simulink model "WBR_control"  (R2021b)
settings: Solver=ode4  StartTime=0.0  StopTime=12  FixedStep=1e-4  RelTol=1e-3
undefined symbols (not defined in the file): leg_controller, leg_l1, leg_l2, leg_model, leg_r1, leg_r2, locomotion_controller, param, sigbuilder_block, wheel_l, wheel_r, X, Y, Z
libraries: sm_lib x110, nesl_utility x29, slpidlib x2
(part 1 of 4)
settings Model: SimulationMode=accelerator  Creator=thinkpad  LastModifiedBy=thinkpad
settings OptimizationCC: DefaultUnderspecifiedDataType=single

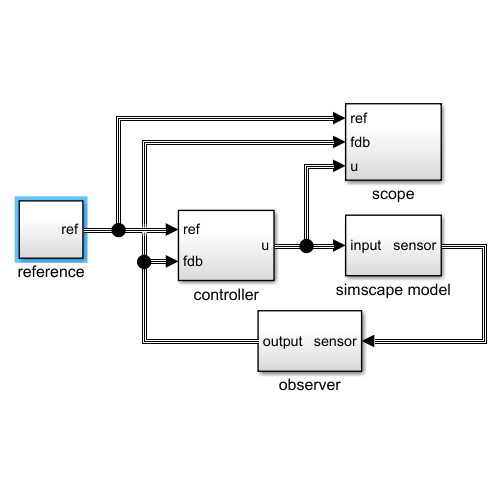
[thumbnail: Simulink's stored preview of the top-level diagram]
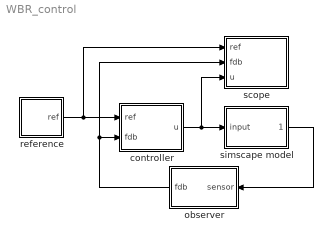
== system WBR_control ==
  controller : Subsystem
  observer : Subsystem
  reference : Subsystem
  scope : Subsystem
  simscape model : Subsystem
  wires:
  reference/1(ref) -> scope/1(ref), controller/1(ref)
  controller/1(u) -> simscape model/1(input), scope/3(u)
  simscape model/1(sensor) -> observer/1(sensor)
  observer/1(fdb) -> controller/2(fdb), scope/2(fdb)

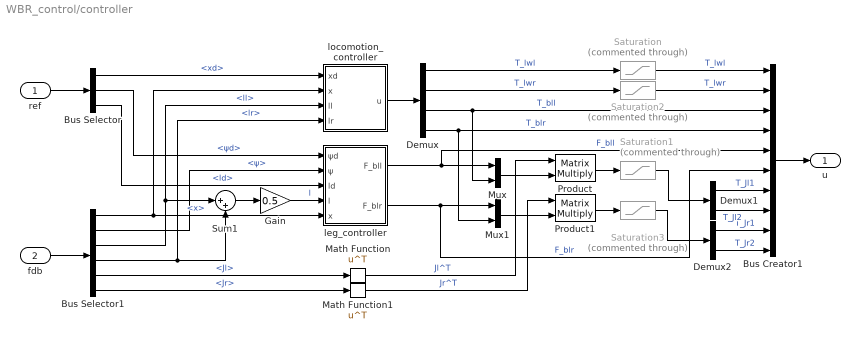
== system WBR_control/controller ==
  ref : Inport
  fdb : Inport  Port=2
  Bus Creator1 : BusCreator  Inputs=10
  Bus Selector : BusSelector  OutputSignals=xd,ψd,ld
  Bus Selector1 : BusSelector  OutputSignals=x,ψ,ll,lr,Jl,Jr
  Demux : Demux
  Demux1 : Demux  Outputs=2
  Demux2 : Demux  Outputs=2
  Gain : Gain  Gain=0.5
  Math Function : Math  Operator=transpose  SaturateOnIntegerOverflow=on
  Math Function1 : Math  Operator=transpose  SaturateOnIntegerOverflow=on
  Mux : Mux  Inputs=2
  Mux1 : Mux  Inputs=2
  Product : Product  Multiplication=Matrix(*)
  Product1 : Product  Multiplication=Matrix(*)
  Saturation : Saturate  Commented=through  UpperLimit=4  LowerLimit=-4
  Saturation1 : Saturate  Commented=through  UpperLimit=[35,35]  LowerLimit=-[35,35]
  Saturation2 : Saturate  Commented=through  UpperLimit=4  LowerLimit=-4
  Saturation3 : Saturate  Commented=through  UpperLimit=[35,35]  LowerLimit=-[35,35]
  Sum1 : Sum  Inputs=|++
  leg_controller : Subsystem
  locomotion_controller : Subsystem
  u : Outport
  wires:
  Bus Selector/1 -> locomotion_controller/1(xd)  "<xd>"
  locomotion_controller/1(u) -> Demux/1
  Demux/1 -> Saturation/1  "T_lwl"
  leg_controller/1(F_bll) -> Bus Creator1/5, Mux/1  "F_bll"
  Bus Selector/2 -> leg_controller/1(ψd)  "<ψd>"
  Bus Selector/3 -> leg_controller/3(ld)  "<ld>"
  Mux/1 -> Product/2
  Product/1 -> Saturation1/1
  ref/1 -> Bus Selector/1
  fdb/1 -> Bus Selector1/1
  Bus Selector1/1 -> locomotion_controller/2(x), leg_controller/5(x)  "<x>"
  Bus Selector1/3 -> locomotion_controller/3(ll), Sum1/1  "<ll>"
  Bus Selector1/4 -> locomotion_controller/4(lr), Sum1/2  "<lr>"
  Bus Selector1/5 -> Math Function/1  "<Jl>"
  Math Function/1 -> Product/1  "Jl^T"
  Demux/2 -> Saturation2/1  "T_lwr"
  Sum1/1 -> Gain/1
  Gain/1 -> leg_controller/4(l)  "l"
  Bus Selector1/6 -> Math Function1/1  "<Jr>"
  Demux/3 -> Mux/2, Bus Creator1/3  "T_bll"
  Demux/4 -> Mux1/2, Bus Creator1/4  "T_blr"
  leg_controller/2(F_blr) -> Bus Creator1/6, Mux1/1  "F_blr"
  Math Function1/1 -> Product1/1  "Jr^T"
  Mux1/1 -> Product1/2
  Product1/1 -> Saturation3/1
  Saturation1/1 -> Demux1/1
  Saturation3/1 -> Demux2/1
  Saturation2/1 -> Bus Creator1/2  "T_lwr"
  Saturation/1 -> Bus Creator1/1  "T_lwl"
  Demux2/1 -> Bus Creator1/9  "T_Jr1"
  Demux2/2 -> Bus Creator1/10  "T_Jr2"
  Demux1/1 -> Bus Creator1/7  "T_Jl1"
  Demux1/2 -> Bus Creator1/8  "T_Jl2"
  Bus Creator1/1 -> u/1
  Bus Selector1/2 -> leg_controller/2(ψ)  "<ψ>"

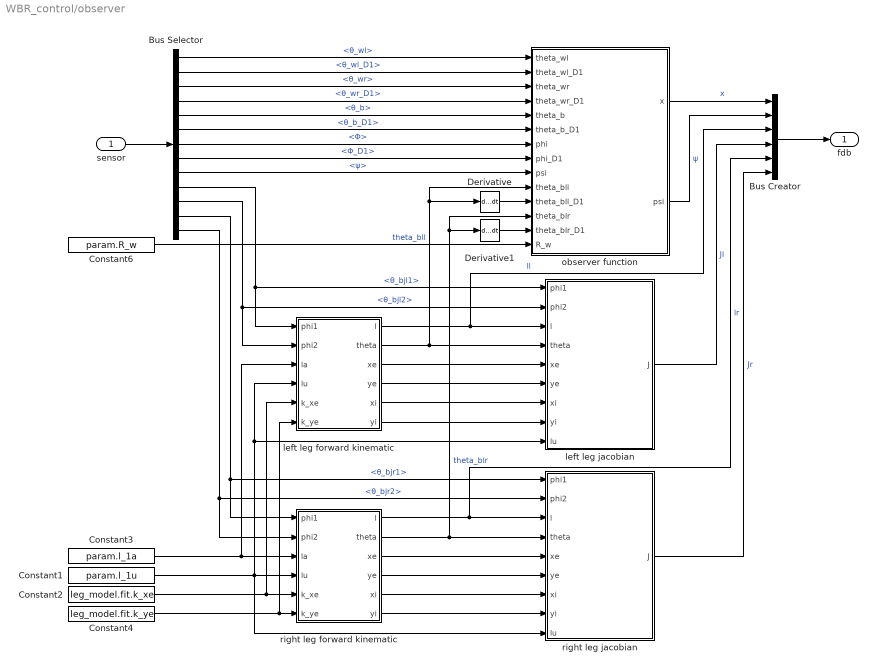
== system WBR_control/observer ==
  sensor : Inport
  Bus Creator : BusCreator  Inputs=6
  Bus Selector : BusSelector  OutputSignals=θ_wl,θ_wl_D1,θ_wr,θ_wr_D1,θ_b,θ_b_D1,Φ,Φ_D1,ψ,θ_bjl1,θ_bjl2,θ_bjr1,θ_bjr2
  Constant1 : Constant  Value=param.l_1u
  Constant2 : Constant  Value=leg_model.fit.k_xe
  Constant3 : Constant  Value=param.l_1a
  Constant4 : Constant  Value=leg_model.fit.k_ye
  Constant6 : Constant  Value=param.R_w
  Derivative : Derivative
  Derivative1 : Derivative
  left leg forward kinematic : MATLAB Function  TreatAsAtomicUnit=on
  left leg jacobian : MATLAB Function  TreatAsAtomicUnit=on
  observer function : MATLAB Function  TreatAsAtomicUnit=on
  right leg forward kinematic : MATLAB Function  TreatAsAtomicUnit=on
  right leg jacobian : MATLAB Function  TreatAsAtomicUnit=on
  fdb : Outport
  wires:
  sensor/1 -> Bus Selector/1
  right leg forward kinematic/3(xe) -> right leg jacobian/5(xe)
  right leg forward kinematic/4(ye) -> right leg jacobian/6(ye)
  right leg forward kinematic/5(xi) -> right leg jacobian/7(xi)
  right leg forward kinematic/6(yi) -> right leg jacobian/8(yi)
  right leg forward kinematic/1(l) -> right leg jacobian/3(l), Bus Creator/5  "lr"
  left leg forward kinematic/1(l) -> Bus Creator/3, left leg jacobian/3(l)  "ll"
  Bus Creator/1 -> fdb/1
  right leg jacobian/1(J) -> Bus Creator/6  "Jr"
  Bus Selector/1 -> observer function/1(theta_wl)  "<θ_wl>"
  Bus Selector/2 -> observer function/2(theta_wl_D1)  "<θ_wl_D1>"
  Bus Selector/3 -> observer function/3(theta_wr)  "<θ_wr>"
  Bus Selector/4 -> observer function/4(theta_wr_D1)  "<θ_wr_D1>"
  Bus Selector/5 -> observer function/5(theta_b)  "<θ_b>"
  Bus Selector/6 -> observer function/6(theta_b_D1)  "<θ_b_D1>"
  Bus Selector/7 -> observer function/7(phi)  "<Φ>"
  Bus Selector/8 -> observer function/8(phi_D1)  "<Φ_D1>"
  left leg jacobian/1(J) -> Bus Creator/4  "Jl"
  observer function/1(x) -> Bus Creator/1  "x"
  observer function/2(psi) -> Bus Creator/2  "ψ"
  Bus Selector/9 -> observer function/9("psi ")  "<ψ>"
  Bus Selector/10 -> left leg forward kinematic/1(phi1), left leg jacobian/1(phi1)  "<θ_bjl1>"
  Bus Selector/11 -> left leg forward kinematic/2(phi2), left leg jacobian/2(phi2)  "<θ_bjl2>"
  left leg forward kinematic/2(theta) -> observer function/10(theta_bll), Derivative/1, left leg jacobian/4(theta)  "theta_bll"
  Derivative/1 -> observer function/11(theta_bll_D1)
  Bus Selector/12 -> right leg jacobian/1(phi1), right leg forward kinematic/1(phi1)  "<θ_bjr1>"
  Bus Selector/13 -> right leg jacobian/2(phi2), right leg forward kinematic/2(phi2)  "<θ_bjr2>"
  right leg forward kinematic/2(theta) -> right leg jacobian/4(theta), observer function/12(theta_blr), Derivative1/1  "theta_blr"
  Derivative1/1 -> observer function/13(theta_blr_D1)
  left leg forward kinematic/4(ye) -> left leg jacobian/6(ye)
  left leg forward kinematic/5(xi) -> left leg jacobian/7(xi)
  left leg forward kinematic/6(yi) -> left leg jacobian/8(yi)
  left leg forward kinematic/3(xe) -> left leg jacobian/5(xe)
  Constant3/1 -> left leg forward kinematic/3(la), right leg forward kinematic/3(la)
  Constant1/1 -> right leg forward kinematic/4(lu), right leg jacobian/9(lu), left leg forward kinematic/4(lu), left leg jacobian/9(lu)
  Constant2/1 -> left leg forward kinematic/5(k_xe), right leg forward kinematic/5(k_xe)
  Constant4/1 -> left leg forward kinematic/6(k_ye), right leg forward kinematic/6(k_ye)
  Constant6/1 -> observer function/14(R_w)

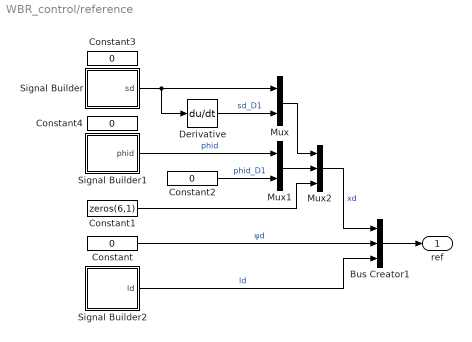
== system WBR_control/reference ==
  Bus Creator1 : BusCreator  Inputs=3
  Constant{,2..4} (4 alike) : Constant  Value=0
  Constant1 : Constant  Value=zeros(6,1)
  Derivative : Derivative
  Mux : Mux  Inputs=2
  Mux1 : Mux  Inputs=2
  Mux2 : Mux  Inputs=3
  Signal Builder : Subsystem  Tag=STV Subsys  LoadFcn=sigbuilder_block('load');  StartFcn=sigbuilder_block('start');  StopFcn=sigbuilder_block('stop');  ClipboardFcn=sigbuilder_block('clipboard');  mask(Sigbuilder block){tuvar=[0:10]}
      mask help: Simulink:masks:SigbuilderBlock_MD
      mask init:
      | if ~strcmp(get_param(bdroot(gcbh),'SimulationStatus'),'stopped') tuvar = sigbuilder_block('maskInit'); end
      settings: CopyFcn=sigbuilder_block('copy');  DeleteFcn=sigbuilder_block('delete');  ModelCloseFcn=sigbuilder_block('modelClose');  PreSaveFcn=sigbuilder_block('preSave');  PauseFcn=sigbuilder_block('pause');  ContinueFcn=sigbuilder_block('continue');  NameChangeFcn=sigbuilder_block('namechange');  OpenFcn=sigbuilder_block('open',[427.2 154.8 550.8 400.2 ]);  CloseFcn=sigbuilder_block('close');
      mask Display: plot(0, 0, 100, 100,[2, 2, 32, 32, 2], [68, 8, 8, 68, 68],[32, 2], [38, 38], [32, 19, 2],[53, 60, 44], [32, 17, 17, 2],[16, 16, 31, 31]);txt = getActiveGroup(gcbh);text(2, 100, txt,'verticalAlignment', 'top');
  Signal Builder1 : Subsystem  Tag=STV Subsys  LoadFcn=sigbuilder_block('load');  StartFcn=sigbuilder_block('start');  StopFcn=sigbuilder_block('stop');  ClipboardFcn=sigbuilder_block('clipboard');  mask(Sigbuilder block){tuvar=[0:10]}
      mask help: Simulink:masks:SigbuilderBlock_MD
      mask init:
      | if ~strcmp(get_param(bdroot(gcbh),'SimulationStatus'),'stopped') tuvar = sigbuilder_block('maskInit'); end
      settings: CopyFcn=sigbuilder_block('copy');  DeleteFcn=sigbuilder_block('delete');  ModelCloseFcn=sigbuilder_block('modelClose');  PreSaveFcn=sigbuilder_block('preSave');  PauseFcn=sigbuilder_block('pause');  ContinueFcn=sigbuilder_block('continue');  NameChangeFcn=sigbuilder_block('namechange');  OpenFcn=sigbuilder_block('open',[427.2 154.8 550.8 400.2 ]);  CloseFcn=sigbuilder_block('close');
      mask Display: plot(0, 0, 100, 100,[2, 2, 32, 32, 2], [68, 8, 8, 68, 68],[32, 2], [38, 38], [32, 19, 2],[53, 60, 44], [32, 17, 17, 2],[16, 16, 31, 31]);txt = getActiveGroup(gcbh);text(2, 100, txt,'verticalAlignment', 'top');
  Signal Builder2 : Subsystem  Tag=STV Subsys  LoadFcn=sigbuilder_block('load');  StartFcn=sigbuilder_block('start');  StopFcn=sigbuilder_block('stop');  ClipboardFcn=sigbuilder_block('clipboard');  mask(Sigbuilder block){tuvar=[0:10]}
      mask help: Simulink:masks:SigbuilderBlock_MD
      mask init:
      | if ~strcmp(get_param(bdroot(gcbh),'SimulationStatus'),'stopped') tuvar = sigbuilder_block('maskInit'); end
      settings: CopyFcn=sigbuilder_block('copy');  DeleteFcn=sigbuilder_block('delete');  ModelCloseFcn=sigbuilder_block('modelClose');  PreSaveFcn=sigbuilder_block('preSave');  PauseFcn=sigbuilder_block('pause');  ContinueFcn=sigbuilder_block('continue');  NameChangeFcn=sigbuilder_block('namechange');  OpenFcn=sigbuilder_block('open',[427.2 154.8 550.8 400.2 ]);  CloseFcn=sigbuilder_block('close');
      mask Display: plot(0, 0, 100, 100,[2, 2, 32, 32, 2], [68, 8, 8, 68, 68],[32, 2], [38, 38], [32, 19, 2],[53, 60, 44], [32, 17, 17, 2],[16, 16, 31, 31]);txt = getActiveGroup(gcbh);text(2, 100, txt,'verticalAlignment', 'top');
  ref : Outport
  wires:
  Mux2/1 -> Bus Creator1/1  "xd"
  Constant1/1 -> Mux2/3
  Signal Builder/1(sd) -> Derivative/1, Mux/1
  Bus Creator1/1 -> ref/1
  Constant2/1 -> Mux1/2  "phid_D1"
  Constant/1 -> Bus Creator1/2  "ψd"
  Mux/1 -> Mux2/1
  Mux1/1 -> Mux2/2
  Signal Builder2/1(ld) -> Bus Creator1/3  "ld"
  Derivative/1 -> Mux/2  "sd_D1"
  Signal Builder1/1(phid) -> Mux1/1  "phid"

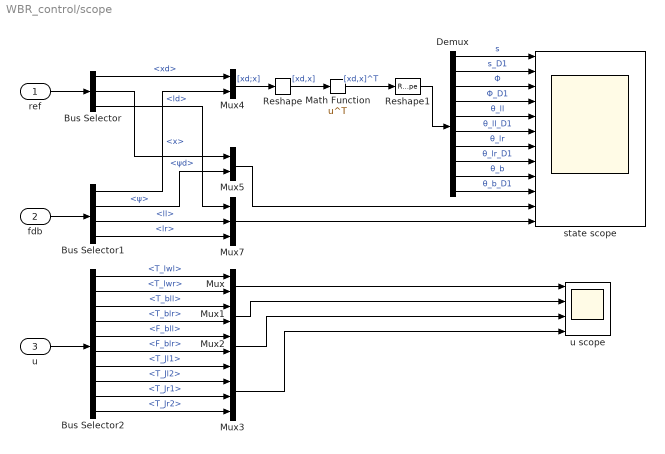
== system WBR_control/scope ==
  ref : Inport
  fdb : Inport  Port=2
  u : Inport  Port=3
  Bus Selector : BusSelector  OutputSignals=xd,ψd,ld
  Bus Selector1 : BusSelector  OutputSignals=x,ψ,ll,lr
  Bus Selector2 : BusSelector  OutputSignals=T_lwl,T_lwr,T_bll,T_blr,F_bll,F_blr,T_Jl1,T_Jl2,T_Jr1,T_Jr2
  Demux : Demux  Outputs=10
  Math Function : Math  Operator=transpose  SaturateOnIntegerOverflow=on
  Mux{,1..2,4..5} (5 alike) : Mux  Inputs=2
  Mux3 : Mux
  Mux7 : Mux  Inputs=3
  Reshape : Reshape  OutputDimensionality=Customize  OutputDimensions=[10,2]
  Reshape1 : Reshape
  state scope : Scope  NumInputPorts=12
  u scope : Scope  NumInputPorts=4
  wires:
  ref/1 -> Bus Selector/1
  fdb/1 -> Bus Selector1/1
  u/1 -> Bus Selector2/1
  Bus Selector2/1 -> Mux/1  "<T_lwl>"
  Bus Selector2/2 -> Mux/2  "<T_lwr>"
  Bus Selector2/3 -> Mux1/1  "<T_bll>"
  Bus Selector2/4 -> Mux1/2  "<T_blr>"
  Bus Selector2/5 -> Mux2/1  "<F_bll>"
  Bus Selector2/6 -> Mux2/2  "<F_blr>"
  Bus Selector2/7 -> Mux3/1  "<T_Jl1>"
  Bus Selector2/8 -> Mux3/2  "<T_Jl2>"
  Bus Selector2/9 -> Mux3/3  "<T_Jr1>"
  Bus Selector2/10 -> Mux3/4  "<T_Jr2>"
  Mux3/1 -> u scope/4
  Mux2/1 -> u scope/3
  Mux1/1 -> u scope/2
  Mux/1 -> u scope/1
  Bus Selector1/1 -> Mux4/2  "<x>"
  Bus Selector/1 -> Mux4/1  "<xd>"
  Bus Selector/2 -> Mux5/1  "<ψd>"
  Bus Selector/3 -> Mux7/1  "<ld>"
  Bus Selector1/2 -> Mux5/2  "<ψ>"
  Bus Selector1/3 -> Mux7/2  "<ll>"
  Bus Selector1/4 -> Mux7/3  "<lr>"
  Mux4/1 -> Reshape/1  "[xd;x]"
  Mux5/1 -> state scope/11
  Mux7/1 -> state scope/12
  Reshape/1 -> Math Function/1  "[xd,x]"
  Math Function/1 -> Reshape1/1  "[xd,x]^T"
  Reshape1/1 -> Demux/1
  Demux/1 -> state scope/1  "s"
  Demux/2 -> state scope/2  "s_D1"
  Demux/3 -> state scope/3  "Φ"
  Demux/4 -> state scope/4  "Φ_D1"
  Demux/6 -> state scope/6  "θ_ll_D1"
  Demux/5 -> state scope/5  "θ_ll"
  Demux/7 -> state scope/7  "θ_lr"
  Demux/8 -> state scope/8  "θ_lr_D1"
  Demux/10 -> state scope/10  "θ_b_D1"
  Demux/9 -> state scope/9  "θ_b"

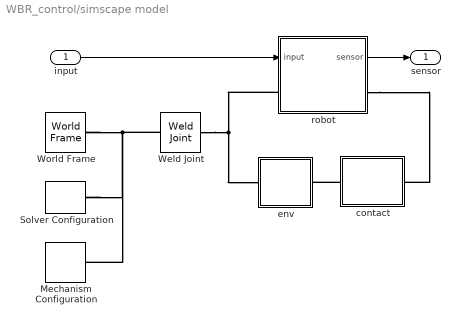
== system WBR_control/simscape model ==
  input : Inport
  Mechanism Configuration : sm_lib/Utilities/Mechanism Configuration  UniformGravity=Constant  GravityVector=[0 0 -9.81]  GravityUnits=m/s^2  LinearizationDelta=0.001  JointModeTransitionNonlinearIterations=2
  Solver Configuration : nesl_utility/Solver Configuration  PhysicalDomain=network_engine_domain  SubClassName=solver  LeftPortType=input  RightPortType=generic  Tones=[]  Harmonics=[]  SimulateNoise=off  Profile=off  UseLocalSampling=off  EnableSwitchedLinearOptims=on  FrequencyDomain=off  UseCCode=off  RelTol=0.001  AbsTol=1e-06  MinStep=1e-09  ToWorkspace=off  RevertToSquareIcSolve=off  NumHomotopyIterations=100  PhasorMode=off  PhasorModeNumHarmonics=1  DoDC=off  ResidualTolerance=1e-09  UseLocalSolver=off  LocalSolverChoice=NE_BACKWARD_EULER_ADVANCER  LocalSolverSampleTime=0.001  DoFixedCost=off  MaxNonlinIter=3  MaxModeIter=2  ComputeImpulses=off  ImpulseIterations=2  LinearAlgebra=Sparse  EquationFormulation=NE_TIME_EF  DelaysMemoryBudget=1024  AutomaticFiltering=on  FilteringTimeConstant=0.001  PartitionStorageMethod=AS_NEEDED  PartitionMemoryBudget=1024  PartitionMethod=FAST
      settings: SourceProductBaseCode=PW,SS
  Weld Joint : sm_lib/Joints/Weld Joint  JointMode=Normal  SenseConstraintForce=off  SenseConstraintForceX=off  SenseConstraintForceY=off  SenseConstraintForceZ=off  SenseConstraintTorque=off  SenseConstraintTorqueX=off  SenseConstraintTorqueY=off  SenseConstraintTorqueZ=off  SenseTotalForce=off  SenseTotalForceX=off  SenseTotalForceY=off  SenseTotalForceZ=off  SenseTotalTorque=off  SenseTotalTorqueX=off  SenseTotalTorqueY=off  SenseTotalTorqueZ=off  CompositeWrenchDir=FollowerOnBase  CompositeWrenchFrame=BaseFrame
  World Frame : sm_lib/Frames and Transforms/World Frame
  contact : Subsystem
      settings: PortSchema="{\"entries\":[{\"content\":{\"sides\":[{\"content\":{\"connectorIds\":[]},\"type\":\"ConnectorPlacement.EquallySpacedRectSide\",\"uuid\":\"948d884d-a2bb-4982-bec2-8891ab05edb1\"},{\"content\":{\"connectorIds\":[],\"side\":\"RIGHT\"},\"type\":\"ConnectorPlacement.EquallySpacedRectSide\",\"uuid\":\"1ab48329-b8c1-41fb-bc52-c8a32a07fc10\"},{\"content\":{\"connectorIds\":[\"LConn1\"],\"side\":\"TOP\"},\"type\":\"ConnectorPlacement.EquallySpacedRectSide\",\"uuid\":\"2430d379-17bc-45a7-9277-8300fd306697\"},{\"content\":{\"connectorIds\":[\"RConn1\"],\"side\":\"BOTTOM\"},\"type\":\"ConnectorPlacement.EquallySpacedRectSide\",\"uuid\":\"c2c22df6-47ef-4364-9ed6-2fe5d2ebd561\"}]},\"type\":\"ConnectorPlacement.EquallySpacedConnector\",\"uuid\":\"bd96c317-3050-474a-affa-ffce42783eb1\"}],\"packageUris\":[\"http://schema.mathworks.com/mf0/Connector/R2020b\"],\"version\":\"1.0\"}"
  env : Subsystem
  robot : Subsystem
  sensor : Outport
  wires:
  input/1 -> robot/1(input)
  robot/1(sensor) -> sensor/1
  connections:
  World Frame/RConn1 -- Solver Configuration/RConn1 -- Mechanism Configuration/RConn1 -- Weld Joint/LConn1
  contact/RConn1 -- env/RConn1
  Weld Joint/RConn1 -- env/LConn1 -- robot/LConn1
  robot/RConn1 -- contact/LConn1

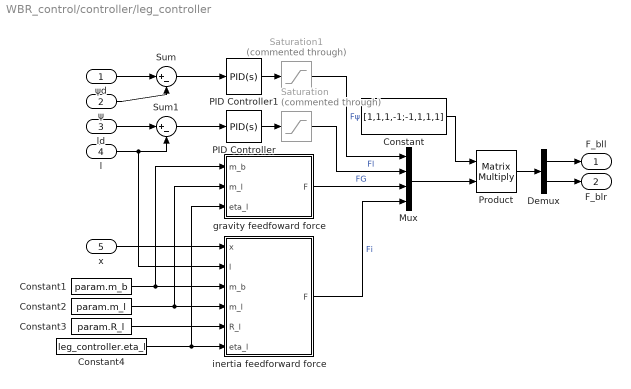
== system WBR_control/controller/leg_controller ==
  ψd : Inport
  ψ : Inport  Port=2
  ld : Inport  Port=3
  l : Inport  Port=4
  x : Inport  Port=5
  Constant : Constant  Value=[1,1,1,-1;-1,1,1,1]
  Constant1 : Constant  Value=param.m_b
  Constant2 : Constant  Value=param.m_l
  Constant3 : Constant  Value=param.R_l
  Constant4 : Constant  Value=leg_controller.eta_l
  Demux : Demux  Outputs=2
  Mux : Mux
  PID Controller : slpidlib/PID Controller  Controller=PID  Form=Parallel  TimeDomain=Continuous-time  UseExternalTs=off  SampleTime=-1  IntegratorMethod=Forward Euler  FilterMethod=Forward Euler  ControllerParametersSource=internal  P=leg_controller.l.kp  I=leg_controller.l.ki  D=leg_controller.l.kd  UseFilter=on  N=100  TunerSelectOption=Transfer Function Based (PID Tuner App)  InitialConditionSource=internal  InitialConditionForIntegrator=0  InitialConditionForFilter=0  DifferentiatorICPrevScaledInput=0  ExternalReset=none  TrackingMode=off  Kt=1  LimitOutput=off  SatLimitsSource=internal  UpperSaturationLimit=inf  LowerSaturationLimit=-inf  LinearizeAsGain=on  AntiWindupMode=none  Kb=1  POutMin=[]  POutMax=[]  IOutMin=[]  IOutMax=[]  DOutMin=[]  DOutMax=[]  NOutMin=[]  NOutMax=[]  SumOutMin=[]  SumOutMax=[]  SaturationOutMin=[]  SaturationOutMax=[]  PParamMin=[]  PParamMax=[]  IParamMin=[]  IParamMax=[]  DParamMin=[]  DParamMax=[]  NParamMin=[]  NParamMax=[]  KbParamMin=[]  KbParamMax=[]  KtParamMin=[]  KtParamMax=[]  KbOutMin=[]  KbOutMax=[]  KtOutMin=[]  KtOutMax=[]  IntegratorOutMin=[]  IntegratorOutMax=[]  FilterOutMin=[]  FilterOutMax=[]  SumI1OutMin=[]  SumI1OutMax=[]  SumI2OutMin=[]  SumI2OutMax=[]  SumI3OutMin=[]  SumI3OutMax=[]  SumI4OutMin=[]  SumI4OutMax=[]  SumDOutMin=[]  SumDOutMax=[]  DifferentiatorOutMin=[]  DifferentiatorOutMax=[]  FilterDiffOutCoefMin=[]  FilterDiffOutCoefMax=[]  ReciprocalOutMin=[]  ReciprocalOutMax=[]  SumDenOutMin=[]  SumDenOutMax=[]  SumNumOutMin=[]  SumNumOutMax=[]  DivideOutMin=[]  DivideOutMax=[]  UdiffTsProdOutMin=[]  UdiffTsProdOutMax=[]  NTsProdOutMin=[]  NTsProdOutMax=[]  UintegralTsProdOutMin=[]  UintegralTsProdOutMax=[]  UngainTsProdOutMin=[]  UngainTsProdOutMax=[]  IntegratorContinuousStateAttributes=''  IntegratorStateMustResolveToSignalObject=off  IntegratorRTWStateStorageClass=Auto  FilterContinuousStateAttributes=''  FilterStateMustResolveToSignalObject=off  FilterRTWStateStorageClass=Auto  ParallelPVariant=InternalParameters  IdealPVariant=Disabled  IVariant=InternalParameters  DVariant=InternalParameters  IntegratorVariant=Continuous  SatVariant=Disabled  AWVariant=Passthrough  PCopyVariant=Disabled  TRVariant=Disabled  FdbkBlocksVariant=Forward  IdealPFdbkVariant=Disabled  SatFdbkVariant=Disabled  DerivativeFilterVariant=ContFilter  NVariant=InternalParameters  NCopyVariant=Disabled  FilterICVariant=InternalICsFilter  IntegratorICVariant=InternalICs  ExternalResetVariant=Disabled  TRSumVariant=Passthrough  SumFdbkVariant=Disabled  SumVariant=Sum_PID  TsampFilterVariant=InternalTs  TsampNgainVariant=Passthrough  TsampIntegralVariant=Passthrough  ExternalSaturationOutDataTypeStr=Inherit: Same as second input
  PID Controller1 : slpidlib/PID Controller  Controller=PID  Form=Parallel  TimeDomain=Continuous-time  UseExternalTs=off  SampleTime=-1  IntegratorMethod=Forward Euler  FilterMethod=Forward Euler  ControllerParametersSource=internal  P=leg_controller.psi.kp  I=leg_controller.psi.ki  D=leg_controller.psi.kd  UseFilter=on  N=100  TunerSelectOption=Transfer Function Based (PID Tuner App)  InitialConditionSource=internal  InitialConditionForIntegrator=0  InitialConditionForFilter=0  DifferentiatorICPrevScaledInput=0  ExternalReset=none  TrackingMode=off  Kt=1  LimitOutput=off  SatLimitsSource=internal  UpperSaturationLimit=inf  LowerSaturationLimit=-inf  LinearizeAsGain=on  AntiWindupMode=none  Kb=1  POutMin=[]  POutMax=[]  IOutMin=[]  IOutMax=[]  DOutMin=[]  DOutMax=[]  NOutMin=[]  NOutMax=[]  SumOutMin=[]  SumOutMax=[]  SaturationOutMin=[]  SaturationOutMax=[]  PParamMin=[]  PParamMax=[]  IParamMin=[]  IParamMax=[]  DParamMin=[]  DParamMax=[]  NParamMin=[]  NParamMax=[]  KbParamMin=[]  KbParamMax=[]  KtParamMin=[]  KtParamMax=[]  KbOutMin=[]  KbOutMax=[]  KtOutMin=[]  KtOutMax=[]  IntegratorOutMin=[]  IntegratorOutMax=[]  FilterOutMin=[]  FilterOutMax=[]  SumI1OutMin=[]  SumI1OutMax=[]  SumI2OutMin=[]  SumI2OutMax=[]  SumI3OutMin=[]  SumI3OutMax=[]  SumI4OutMin=[]  SumI4OutMax=[]  SumDOutMin=[]  SumDOutMax=[]  DifferentiatorOutMin=[]  DifferentiatorOutMax=[]  FilterDiffOutCoefMin=[]  FilterDiffOutCoefMax=[]  ReciprocalOutMin=[]  ReciprocalOutMax=[]  SumDenOutMin=[]  SumDenOutMax=[]  SumNumOutMin=[]  SumNumOutMax=[]  DivideOutMin=[]  DivideOutMax=[]  UdiffTsProdOutMin=[]  UdiffTsProdOutMax=[]  NTsProdOutMin=[]  NTsProdOutMax=[]  UintegralTsProdOutMin=[]  UintegralTsProdOutMax=[]  UngainTsProdOutMin=[]  UngainTsProdOutMax=[]  IntegratorContinuousStateAttributes=''  IntegratorStateMustResolveToSignalObject=off  IntegratorRTWStateStorageClass=Auto  FilterContinuousStateAttributes=''  FilterStateMustResolveToSignalObject=off  FilterRTWStateStorageClass=Auto  ParallelPVariant=InternalParameters  IdealPVariant=Disabled  IVariant=InternalParameters  DVariant=InternalParameters  IntegratorVariant=Continuous  SatVariant=Disabled  AWVariant=Passthrough  PCopyVariant=Disabled  TRVariant=Disabled  FdbkBlocksVariant=Forward  IdealPFdbkVariant=Disabled  SatFdbkVariant=Disabled  DerivativeFilterVariant=ContFilter  NVariant=InternalParameters  NCopyVariant=Disabled  FilterICVariant=InternalICsFilter  IntegratorICVariant=InternalICs  ExternalResetVariant=Disabled  TRSumVariant=Passthrough  SumFdbkVariant=Disabled  SumVariant=Sum_PID  TsampFilterVariant=InternalTs  TsampNgainVariant=Passthrough  TsampIntegralVariant=Passthrough  ExternalSaturationOutDataTypeStr=Inherit: Same as second input
  Product : Product  Multiplication=Matrix(*)
  Saturation : Saturate  Commented=through  UpperLimit=30  LowerLimit=-30
  Saturation1 : Saturate  Commented=through  UpperLimit=30  LowerLimit=-30
  Sum : Sum  Inputs=|+-
  Sum1 : Sum  Inputs=|+-
  gravity feedfoward force : MATLAB Function  TreatAsAtomicUnit=on
  inertia feedforward force : MATLAB Function  TreatAsAtomicUnit=on
  F_bll : Outport
  F_blr : Outport  Port=2
  wires:
  ψ/1 -> Sum/2
  l/1 -> inertia feedforward force/2(l), Sum1/2
  ld/1 -> Sum1/1
  ψd/1 -> Sum/1
  Sum1/1 -> PID Controller/1
  Sum/1 -> PID Controller1/1
  PID Controller1/1 -> Saturation1/1
  PID Controller/1 -> Saturation/1
  Saturation1/1 -> Mux/1  "Fψ"
  Saturation/1 -> Mux/2  "Fl"
  x/1 -> inertia feedforward force/1(x)
  gravity feedfoward force/1(F) -> Mux/3  "FG"
  inertia feedforward force/1(F) -> Mux/4  "Fi"
  Mux/1 -> Product/2
  Constant/1 -> Product/1
  Product/1 -> Demux/1
  Demux/2 -> F_blr/1
  Demux/1 -> F_bll/1
  Constant1/1 -> gravity feedfoward force/1(m_b), inertia feedforward force/3(m_b)
  Constant2/1 -> gravity feedfoward force/2(m_l), inertia feedforward force/4(m_l)
  Constant3/1 -> inertia feedforward force/5(R_l)
  Constant4/1 -> gravity feedfoward force/3(eta_l), inertia feedforward force/6(eta_l)

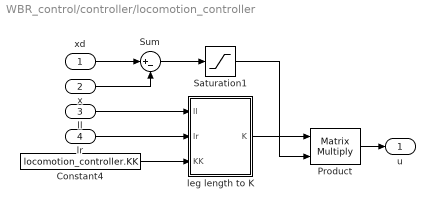
== system WBR_control/controller/locomotion_controller ==
  xd : Inport
  x : Inport  Port=2
  ll : Inport  Port=3
  lr : Inport  Port=4
  Constant4 : Constant  Value=locomotion_controller.KK
  Product : Product  Multiplication=Matrix(*)
  Saturation1 : Saturate  UpperLimit=[0.5,3,0.5*pi,3*pi,inf,inf,inf,inf,inf,inf]'  LowerLimit=-[0.5,3,0.5*pi,3*pi,inf,inf,inf,inf,inf,inf]'
  Sum : Sum  Inputs=|+-
  leg length to K : MATLAB Function  TreatAsAtomicUnit=on
  u : Outport
  wires:
  Product/1 -> u/1
  Saturation1/1 -> Product/2
  leg length to K/1(K) -> Product/1
  ll/1 -> leg length to K/1(ll)
  x/1 -> Sum/2
  xd/1 -> Sum/1
  Sum/1 -> Saturation1/1
  lr/1 -> leg length to K/2(lr)
  Constant4/1 -> leg length to K/3(KK)

== system WBR_control/reference/Signal Builder ==
  Demux : Demux  Tag=STV Demux  Outputs=1
      settings: DisplayOption=none
  FromWs : FromWorkspace  Tag=STV FromWs  VariableName=tuvar
      SigBuilderData=|
      | common.afterFinalStr = 'Extrapolate'
      | common.sampleTime = 0
      | dataSet.timeRange = [0 20]
      | dataSet.name = 'ref'
      | sbobj.Groups.Name = 'ref'
      | sbobj.Groups.Signals.Name = 'sd'
      | sbobj.Groups.Signals.XData = [0 1.5 2 4.5 7 10 20]
      | sbobj.Groups.Signals.YData = [0.1 -3.5 -3.5 4 4 0 0]
      | sbobj.Groups.TimeRange = [0 20]
  sd : Outport  Tag=STV Outport
  wires:
  Demux/1 -> sd/1
  FromWs/1 -> Demux/1

== system WBR_control/reference/Signal Builder1 ==
  Demux : Demux  Tag=STV Demux  Outputs=1
      settings: DisplayOption=none
  FromWs : FromWorkspace  Tag=STV FromWs  VariableName=tuvar
      SigBuilderData=|
      | common.afterFinalStr = 'Extrapolate'
      | common.sampleTime = 0
      | dataSet.timeRange = [0 20]
      | dataSet.name = 'ref'
      | sbobj.Groups.Name = 'ref'
      | sbobj.Groups.Signals.Name = 'phid'
      | sbobj.Groups.Signals.XData = [0 1.5 4.5 5 8 11 20]
      | sbobj.Groups.Signals.YData = [0 0 0 1.57079632679 1.57079632679 0 0]
      | sbobj.Groups.TimeRange = [0 20]
  phid : Outport  Tag=STV Outport
  wires:
  Demux/1 -> phid/1
  FromWs/1 -> Demux/1

== system WBR_control/reference/Signal Builder2 ==
  Demux : Demux  Tag=STV Demux  Outputs=1
      settings: DisplayOption=none
  FromWs : FromWorkspace  Tag=STV FromWs  VariableName=tuvar
      SigBuilderData=|
      | common.afterFinalStr = 'Extrapolate'
      | common.sampleTime = 0
      | dataSet.timeRange = [0 20]
      | dataSet.name = 'ref'
      | sbobj.Groups.Name = 'ref'
      | sbobj.Groups.Signals.Name = 'ld'
      | sbobj.Groups.Signals.XData = [0 4 8 12 20]
      | sbobj.Groups.Signals.YData = [0.25 0.25 0.25 0.25 0.25]
      | sbobj.Groups.TimeRange = [0 20]
  ld : Outport  Tag=STV Outport
  wires:
  Demux/1 -> ld/1
  FromWs/1 -> Demux/1

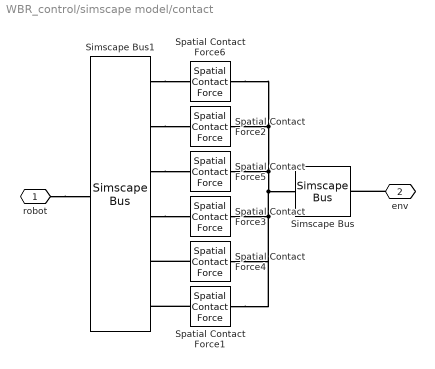
== system WBR_control/simscape model/contact ==
  Simscape Bus : SimscapeBus  HierarchyStrings=ground
  Simscape Bus1 : SimscapeBus  HierarchyStrings=leg_l1;leg_l2;leg_r1;leg_r2;wheel_l;wheel_r
  Spatial Contact Force1 : sm_lib/Forces and Torques/Spatial Contact Force  CoefficientOfDynamicFriction=0.3  CoefficientOfStaticFriction=0.5  SenseContactBaseRotation=off  SenseContactBaseTranslation=off  NormalDamping=1e5  NormalDampingUnits=N/(m/s)  SenseContactFollowerRotation=off  SenseContactFollowerTranslation=off  SenseContactSignal=off  NormalStiffness=1e6  NormalStiffnessUnits=N/m  FrictionalCriticalVelocity=1e-3  FrictionalCriticalVelocityUnits=m/s  ZeroCrossDetectContactStartAndEnd=off  FrictionType=SmoothStickSlip  SenseFrictionalForceMagnitude=off  SenseNormalForceMagnitude=off  NormalForceType=SmoothSpringDamper  SenseNormalVelocity=off  SenseSeparationDistance=off  SenseTangentialVelocity=off  SenseTangentialVelocityMagnitude=off  NormalTransitionRegionWidth=1e-4  NormalTransitionRegionWidthUnits=m
  Spatial Contact Force{2..3,5..6} (4 alike) : sm_lib/Forces and Torques/Spatial Contact Force  CoefficientOfDynamicFriction=0.3  CoefficientOfStaticFriction=0  SenseContactBaseRotation=off  SenseContactBaseTranslation=off  NormalDamping=1e5  NormalDampingUnits=N/(m/s)  SenseContactFollowerRotation=off  SenseContactFollowerTranslation=off  SenseContactSignal=off  NormalStiffness=1e6  NormalStiffnessUnits=N/m  FrictionalCriticalVelocity=1e-3  FrictionalCriticalVelocityUnits=m/s  ZeroCrossDetectContactStartAndEnd=off  FrictionType=SmoothStickSlip  SenseFrictionalForceMagnitude=off  SenseNormalForceMagnitude=off  NormalForceType=SmoothSpringDamper  SenseNormalVelocity=off  SenseSeparationDistance=off  SenseTangentialVelocity=off  SenseTangentialVelocityMagnitude=off  NormalTransitionRegionWidth=1e-4  NormalTransitionRegionWidthUnits=m
  Spatial Contact Force4 : sm_lib/Forces and Torques/Spatial Contact Force  CoefficientOfDynamicFriction=0.3  CoefficientOfStaticFriction=0.5  SenseContactBaseRotation=off  SenseContactBaseTranslation=off  NormalDamping=1e5  NormalDampingUnits=N/(m/s)  SenseContactFollowerRotation=off  SenseContactFollowerTranslation=off  SenseContactSignal=off  NormalStiffness=1e6  NormalStiffnessUnits=N/m  FrictionalCriticalVelocity=1e-3  FrictionalCriticalVelocityUnits=m/s  ZeroCrossDetectContactStartAndEnd=off  FrictionType=SmoothStickSlip  SenseFrictionalForceMagnitude=off  SenseNormalForceMagnitude=off  NormalForceType=SmoothSpringDamper  SenseNormalVelocity=off  SenseSeparationDistance=off  SenseTangentialVelocity=off  SenseTangentialVelocityMagnitude=off  NormalTransitionRegionWidth=1e-4  NormalTransitionRegionWidthUnits=m
  robot : PMIOPort  Side=Left
  env : PMIOPort  Port=2  Side=Right
  connections:
  Spatial Contact Force4/LConn1 -- Simscape Bus1/LConn5
  env/RConn1 -- Simscape Bus/RConn1
  robot/RConn1 -- Simscape Bus1/RConn1
  Simscape Bus1/LConn2 -- Spatial Contact Force2/LConn1
  Spatial Contact Force2/RConn1 -- Spatial Contact Force6/RConn1 -- Spatial Contact Force5/RConn1 -- Spatial Contact Force3/RConn1 -- Spatial Contact Force1/RConn1 -- Spatial Contact Force4/RConn1 -- Simscape Bus/LConn1
  Spatial Contact Force1/LConn1 -- Simscape Bus1/LConn6
  Simscape Bus1/LConn4 -- Spatial Contact Force3/LConn1
  Simscape Bus1/LConn1 -- Spatial Contact Force6/LConn1
  Simscape Bus1/LConn3 -- Spatial Contact Force5/LConn1

== system WBR_control/simscape model/env ==
  Rigid Transform3 : sm_lib/Frames and Transforms/Rigid Transform  TranslationMethod=StandardAxis  TranslationStandardOffset=-0.05  TranslationLengthUnit=m  TranslationStandardAxis=+Z  TranslationCartesianOffset=[0 0 0]  TranslationROffset=0  TranslationROffsetUnits=m  TranslationZOffset=0  TranslationZOffsetUnits=m  TranslationThetaOffset=0  TranslationThetaOffsetUnits=deg  RotationMethod=None  RotationAngleUnits=deg  RotationStandardAxis=+X  RotationAngle=90  RotationArbitraryAxis=[0 0 1]  FollAlignAxisA=+X  BaseAlignAxisA=+Y  FollAlignAxisB=+Y  BaseAlignAxisB=+Z  RotationSequenceAxes=FollowerAxes  RotationSequence=XYX  RotationSequenceAngles=[0 0 0]  RotationSequenceAnglesUnits=deg  RotationMatrix=[1 0 0; 0 1 0; 0 0 1]
  Simscape Bus : SimscapeBus  HierarchyStrings=ground
  ground : sm_lib/Body Elements/Brick Solid  GraphicAmbientColor=[0.15 0.15 0.15 1.0]  BasedOnType=Density  BrickDimensions=[10 10 0.1]  BrickDimensionUnits=m  CenterOfMass=[0 0 0]  CenterOfMassUnits=m  GraphicDiffuseColor=[0.9 0.9 0.9]  Density=1000  DensityUnits=kg/m^3  DoExposeReferenceFrame=on  GraphicEmissiveColor=[0.0 0.0 0.0 1.0]  ExportEntireGeometry=on  SerializedFrames=<Frames/>  MarkerShape=Sphere  MarkerSize=10  GraphicType=FromGeometry  InertiaType=CalculateFromGeometry  Mass=1  MassUnits=kg  MomentsOfInertia=[1 1 1]  MomentsOfInertiaUnits=kg*m^2  GraphicOpacity=1.0  ProductsOfInertia=[0 0 0]  ProductsOfInertiaUnits=kg*m^2  GraphicShininess=75  GraphicSpecularColor=[0.5 0.5 0.5 1.0]  GraphicVisPropType=SimpleVisualProperties
  R : PMIOPort  Side=Left
  G : PMIOPort  Port=2  Side=Right
  connections:
  Simscape Bus/RConn1 -- G/RConn1
  ground/RConn1 -- Rigid Transform3/RConn1
  ground/LConn1 -- Simscape Bus/LConn1
  Rigid Transform3/LConn1 -- R/RConn1
